simulink model "quadrotor_sim"  (R2020b)
settings: Solver=ode4  StartTime=0.0  StopTime=150  FixedStep=0.01  RelTol=1e-3  EnableMultiTasking=on
settings Model: Creator=yubin_000  LastModifiedBy=mikel
settings DataIOCC: LimitDataPoints=on  SaveFormat=Array  SignalLoggingSaveFormat=ModelDataLogs  ReturnWorkspaceOutputs=off
settings OptimizationCC: LifeSpan=inf
settings DebuggingCC: SolverPrmCheckMsg=warning  MultiTaskDSMMsg=warning  MultiTaskCondExecSysMsg=none  StrictBusMsg=ErrorOnBusTreatedAsVector  SFUnexpectedBacktrackingDiag=warning  SFNoUnconditionalDefaultTransitionDiag=warning  SFExecutionAtInitializationDiag=none  ArithmeticOperatorsInVariantConditions=warning
settings HardwareCC: ProdBitPerPointer=32  ProdBitPerSizeT=32  ProdBitPerPtrDiffT=32  ProdLargestAtomicFloat=None  ProdIntDivRoundTo=Undefined  ProdEndianess=Unspecified  ProdWordSize=32  ProdHWDeviceType=32-bit Generic
settings ModelReferenceCC: PropagateSignalLabelsOutOfModel=off
settings SFSimCC: SimUseLocalCustomCode=off  CustomCodeUndefinedFunction=UseInterfaceOnly
settings RTWCC: RTWUseLocalCustomCode=off
settings CodeAppCC: StateflowObjectComments=on
settings GRTTargetCC: TargetLangStandard=C89/C90 (ANSI)
settings ConfigComp: CovMetricSettings=dw  CovSaveCumulativeToWorkspaceVar=on  CovSaveSingleToWorkspaceVar=on  CovExternalEMLEnable=off

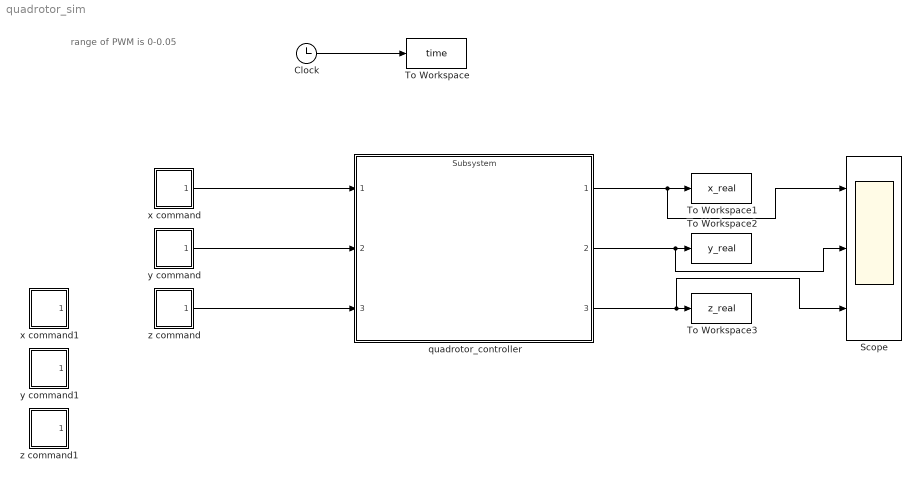
== system quadrotor_sim ==
  note: range of PWM is 0-0.05
  Clock : Clock
  Scope : Scope  NumInputPorts=3
  To Workspace : ToWorkspace  VariableName=time  SampleTime=-1
  To Workspace1 : ToWorkspace  VariableName=x_real  SampleTime=-1
  To Workspace2 : ToWorkspace  VariableName=y_real  SampleTime=-1
  To Workspace3 : ToWorkspace  VariableName=z_real  SampleTime=-1
  quadrotor_controller : ModelReference  ModelNameDialog=Subsystem  ModelReferenceVersion=1.550  CopyOfModelProtected=on
      mask Display: image('434526310377837331.jpg'); % Use "Edit Image" on toolstrip to change.
  x command : Subsystem
  x command1 : Subsystem
  y command : Subsystem
  y command1 : Subsystem
  z command : Subsystem
  z command1 : Subsystem
  wires:
  Clock/1 -> To Workspace/1
  quadrotor_controller/1 -> Scope/1, To Workspace1/1
  quadrotor_controller/2 -> Scope/2, To Workspace2/1
  quadrotor_controller/3 -> Scope/3, To Workspace3/1
  x command/1(Out1) -> quadrotor_controller/1
  y command/1(Out1) -> quadrotor_controller/2
  z command/1(Out1) -> quadrotor_controller/3

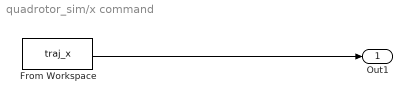
== system quadrotor_sim/x command ==
  From Workspace : FromWorkspace  VariableName=traj_x  SampleTime=0.01  OutputAfterFinalValue=Holding final value
  Out1 : Outport
  wires:
  From Workspace/1 -> Out1/1

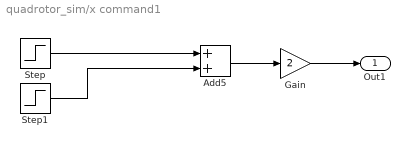
== system quadrotor_sim/x command1 ==
  Add5 : Sum
  Gain : Gain  Gain=2
  Step : Step  Time=10  SampleTime=0
  Step1 : Step  Time=20  After=-1  SampleTime=0
  Out1 : Outport
  wires:
  Gain/1 -> Out1/1
  Step/1 -> Add5/1
  Add5/1 -> Gain/1
  Step1/1 -> Add5/2

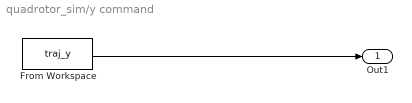
== system quadrotor_sim/y command ==
  From Workspace : FromWorkspace  VariableName=traj_y  SampleTime=0.01  OutputAfterFinalValue=Holding final value
  Out1 : Outport
  wires:
  From Workspace/1 -> Out1/1

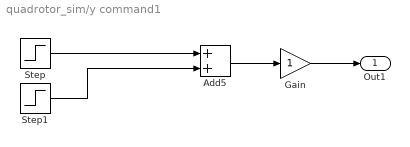
== system quadrotor_sim/y command1 ==
  Add5 : Sum
  Gain : Gain
  Step : Step  Time=10  SampleTime=0
  Step1 : Step  Time=20  After=-1  SampleTime=0
  Out1 : Outport
  wires:
  Step1/1 -> Add5/2
  Add5/1 -> Gain/1
  Step/1 -> Add5/1
  Gain/1 -> Out1/1

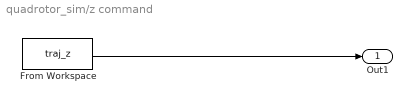
== system quadrotor_sim/z command ==
  From Workspace : FromWorkspace  VariableName=traj_z  SampleTime=0.01  OutputAfterFinalValue=Holding final value
  Out1 : Outport
  wires:
  From Workspace/1 -> Out1/1

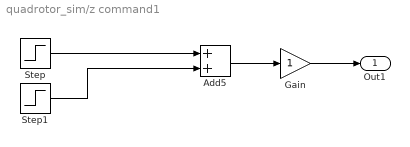
== system quadrotor_sim/z command1 ==
  Add5 : Sum
  Gain : Gain
  Step : Step  Time=10  SampleTime=0
  Step1 : Step  Time=20  After=-1  SampleTime=0
  Out1 : Outport
  wires:
  Gain/1 -> Out1/1
  Step/1 -> Add5/1
  Add5/1 -> Gain/1
  Step1/1 -> Add5/2
